simulink model "sf_debouncer"  (R2025b)
settings: Solver=VariableStepDiscrete  StartTime=0.0  StopTime=6  RelTol=1e-3  EnableMultiTasking=on
settings Model: Creator=The MathWorks, Inc.  LastModifiedBy=The MathWorks, Inc.
settings SolverCC: AlgebraicLoopSolver=TrustRegion  InsertRTBMode=Auto
settings DataIOCC: LimitDataPoints=on  SaveFormat=Array  ReturnWorkspaceOutputs=off
settings OptimizationCC: ReuseModelBlockBuffer=off  ExpressionDepthLimit=2147483647.0  InitFltsAndDblsToZero=on  EfficientMapNaN2IntZero=off  LifeSpan=inf
settings DebuggingCC: SaveWithParameterizedLinksMsg=none  UnderspecifiedInitializationDetection=Classic  MergeDetectMultiDrivingBlocksExec=none  SignalResolutionControl=TryResolveAllWithWarning  SolverPrmCheckMsg=warning  MultiTaskDSMMsg=warning  MultiTaskCondExecSysMsg=none  FcnCallInpInsideContextMsg=warning  UnconnectedInputMsg=warning  UnconnectedOutputMsg=warning  UnconnectedLineMsg=warning  StateNameClashWarn=warning  SFUnexpectedBacktrackingDiag=warning  SFNoUnconditionalDefaultTransitionDiag=warning  SFExecutionAtInitializationDiag=none  ArithmeticOperatorsInVariantConditions=warning
settings HardwareCC: ProdBitPerPointer=32.0  ProdBitPerSizeT=32.0  ProdBitPerPtrDiffT=32.0  ProdLargestAtomicFloat=None  ProdIntDivRoundTo=Undefined  ProdEndianess=Unspecified  ProdWordSize=32.0  ProdHWDeviceType=32-bit Generic
settings ModelReferenceCC: EnableRefExpFcnMdlSchedulingChecks=on  PropagateSignalLabelsOutOfModel=off
settings SFSimCC: SimUseLocalCustomCode=off  SimParseCustomCode=off  CustomCodeUndefinedFunction=UseInterfaceOnly
settings RTWCC: RTWUseLocalCustomCode=off  GPUComputeCapability=3.5
settings CodeAppCC: StateflowObjectComments=on
settings GRTTargetCC: TargetFcnLib=ansi_tfl_tmw.mat  TargetLangStandard=C89/C90 (ANSI)  CombineOutputUpdateFcns=off  GRTInterface=on
settings ConfigComp: CovMetricSettings=dw  CovSaveCumulativeToWorkspaceVar=on  CovSaveSingleToWorkspaceVar=on  CovExternalEMLEnable=off  CovSFcnEnable=off

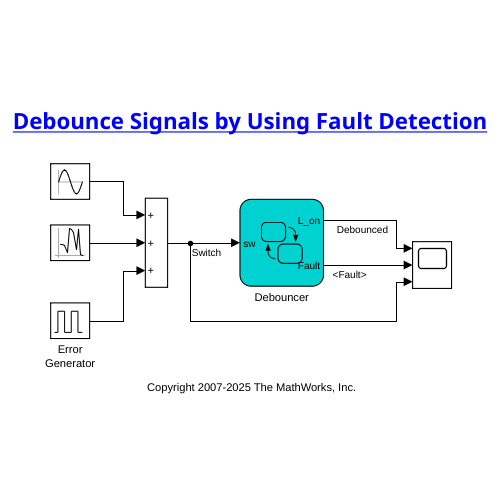
[thumbnail: Simulink's stored preview of the top-level diagram]
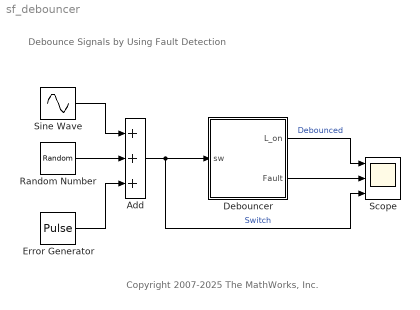
== system sf_debouncer ==
  note: Copyright 2007-2025 The MathWorks, Inc.
  note: Debounce Signals by Using Fault Detection
  Add : Sum  Inputs=+++
  Debouncer : Stateflow chart  TreatAsAtomicUnit=on
  Error Generator : DiscretePulseGenerator  PulseType=Time based  Amplitude=10  Period=0.001  PulseWidth=50  PhaseDelay=2
  Random Number : RandomNumber  Variance=30  SampleTime=0
  Scope : Scope  NumInputPorts=3
      settings: TimeSpan=6.5  ActiveDisplayYMinimum=-1  ActiveDisplayYMaximum=1.5  DataLoggingMaxPoints=10000
  Sine Wave : Sin  Amplitude=20  Frequency=10  SampleTime=0
  wires:
  Debouncer/1(L_on) -> Scope/1  "Debounced"
  Sine Wave/1 -> Add/1
  Random Number/1 -> Add/2
  Add/1 -> Debouncer/1(sw), Scope/3  "Switch"
  Error Generator/1 -> Add/3
  Debouncer/2(" Fault") -> Scope/2

== stateflow chart sf_debouncer/Debouncer ==
  settings: updateMethod=DISCRETE  sampleTime=0.001
  state Off
    en: L_on = 0;
    state Fault
      % Isolation
    state Normal
    Fault -> Normal : % Recovery
        | after(1, sec)
    (default) -> Normal
  state Debounce
    state Off
    state On
    Debounce.Off -> Debounce.On [order 2] : [sw > 0]
    Debounce.On -> Debounce.Off [order 2] : [sw < 0]
  state On
    en: L_on = 1;
  (default) -> Off
  Debounce -> Fault : % Detection
      | after(0.3, sec)
  Normal -> Debounce.On : [sw > 0]
  Debounce.Off -> Off [order 1] : after(0.1, sec)
  On -> Debounce.Off : [sw < 0]
  Debounce.On -> On [order 1] : after(0.1, sec)
  data: sw input; L_on output double; Fault output boolean
